simulink model "vdynblksskidpad_final"  (R2026b)
settings: Solver=ode23t  StopTime=inf  RelTol=5e-3
model workspace (MAT data in the model file):
  Eng : object (value not decoded)
  Nmtr = 11.5
  StartupTrim : object (value not decoded)
  SteerLim = 60
  TrackPoints = [-15 -12 -9 -6 -3 5.58745102111e-16 2.81978007367 5.36354042717 7.38228007367 8.67839071119 9.125 8.67839071119 ... (270 elements, 90x3)]
  Trans : object (value not decoded)
  Ts = 0.02
  VEH : object (value not decoded)
values from neighbouring files (symbols this model uses):
  n = size(e.Data,2)    [plot_skidpad_signals.m]
  z = tsMatrix(out.diagWheel.z)    [skidpad_settle_start.m]
symbols that are objects in the model workspace (value not decoded): Eng, StartupTrim, Trans, VEH
undefined symbols (not defined in the file or in its folder): BdyFrm, InertFrm, magnitude
libraries: autolibsharedcoupling x11, simulink x8, sim3dlib x7, autolibshareddiff x5, autolibutils x4, sim3dautolib x3, vehdynlibtirecommon x3, sharedtransform x3, vehdynlibdriver x2, vehdynlibsteering x2, vehdynlibeom x2, vehdynlibviscommon x2
(part 2 of 5)

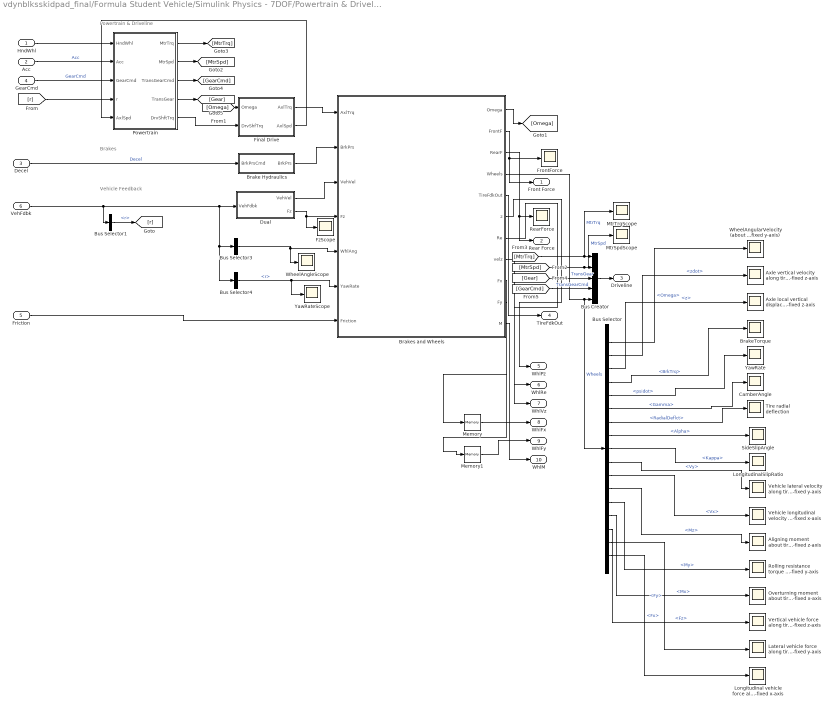
== system vdynblksskidpad_final/Formula Student Vehicle/Simulink Physics - 7DOF/Powertrain & Driveline ==
  note: Brakes
  note: Powertrain & Driveline
  note: Vehicle Feedback
  HndWhl : Inport
  Acc : Inport  Port=2
  Decel : Inport  Port=3
  GearCmd : Inport  Port=4
  Friction : Inport  Port=5
  VehFdbk : Inport  Port=6
  Aligning moment about tire-fixed z-axis : Scope
      settings: DataLoggingVariableName=ScopeData27
  "Axle local vertical displacement along tire-fixed z-axis " : Scope
      settings: DataLoggingVariableName=ScopeData18
  Axle vertical velocity along tire-fixed z-axis : Scope
      settings: DataLoggingVariableName=ScopeData17
  Brake Hydraulics : Subsystem
  BrakeTorque : Scope
      settings: DataLoggingVariableName=ScopeData19
  Brakes and Wheels : Subsystem
      mask Display: image('vdbslibwhls.png');
  Bus Creator : BusCreator  Inputs=5
  Bus Selector : BusSelector  OutputSignals=Omega,zdot,z,BrkTrq,psidot,Gamma,RadialDeflct,Alpha,Kappa,Vy,Vx,Mz,My,Mx,Fz,Fy,Fx
  Bus Selector1 : BusSelector  OutputSignals=signal1.VehFdbk.BdyFrm.Cg.AngVel.r
  Bus Selector3 : BusSelector  OutputSignals=signal2  OutputAsBus=on
  Bus Selector4 : BusSelector  OutputSignals=signal1.VehFdbk.BdyFrm.Cg.AngVel.r
  CamberAngle : Scope
      settings: DataLoggingVariableName=ScopeData21
  Dual : Subsystem  VariantControl=1
  Final Drive : Subsystem  Variant=on  VariantControlMode=label  VariantControl=Variant1  LabelModeActiveChoice=Direct
  FrontForce : Scope
      settings: ActiveDisplayYMinimum=-5430.7562675409335  ActiveDisplayYMaximum=5616.5134549978548  DataLoggingVariableName=ScopeData6
  FzScope : Scope
      settings: ActiveDisplayYMinimum=-645.63329923322237  ActiveDisplayYMaximum=1662.7938538455548  DataLoggingVariableName=ScopeData8
  Lateral vehicle force along tire-fixed y-axis : Scope
      settings: DataLoggingVariableName=ScopeData31
  Longitudinal vehicle force along tire-fixed x-axis : Scope
      settings: DataLoggingVariableName=ScopeData32
  LongitudinalSlipRatio : Scope
      settings: DataLoggingVariableName=ScopeData24
  Memory : Memory
  Memory1 : Memory
  MtrSpdScope : Scope
      settings: ActiveDisplayYMinimum=-7990.9819579860705  ActiveDisplayYMaximum=10917.06072261999  DataLoggingVariableName=ScopeData5
  MtrTrqScope : Scope
      settings: ActiveDisplayYMinimum=-20.850315998209098  ActiveDisplayYMaximum=27.207842066624828  DataLoggingVariableName=ScopeData4
  "Overturning moment about tire-fixed x-axis " : Scope
      settings: DataLoggingVariableName=ScopeData29
  Powertrain : Subsystem  Variant=on  VariantControlMode=label  VariantControl=Powertrain  LabelModeActiveChoice=EV4EM  EmptyChoice=on
  RearForce : Scope
      settings: ActiveDisplayYMinimum=-3774.7383769148314  ActiveDisplayYMaximum=3034.9269366821081  DataLoggingVariableName=ScopeData7
  Rolling resistance torque about tire-fixed y-axis : Scope
      settings: DataLoggingVariableName=ScopeData28
  SideSlipAngle : Scope
      settings: ActiveDisplayYMinimum=-0.025723950583025436  ActiveDisplayYMaximum=-0.012444025446734935  DataLoggingVariableName=ScopeData23
  Tire radial deflection : Scope
      settings: DataLoggingVariableName=ScopeData22
  Vehicle lateral velocity along tire-fixed y-axis : Scope
      settings: DataLoggingVariableName=ScopeData25
  Vehicle longitudinal velocity along tire-fixed x-axis : Scope
      settings: ActiveDisplayYMinimum=-9.3486138693816443  ActiveDisplayYMaximum=18.874913708365771  DataLoggingVariableName=ScopeData26
  Vertical vehicle force along tire-fixed z-axis : Scope
      settings: DataLoggingVariableName=ScopeData30
  WheelAngleScope : Scope
      settings: ActiveDisplayYMinimum=-1.4321699263684977  ActiveDisplayYMaximum=0.32820753202327618  DataLoggingVariableName=ScopeData10
  WheelAngularVelocity (about wheel-fixed y-axis) : Scope
      settings: ActiveDisplayYMinimum=-103.38838312860861  ActiveDisplayYMaximum=88.850056409744354  DataLoggingVariableName=ScopeData16
  YawRate : Scope
      settings: DataLoggingVariableName=ScopeData20
  YawRateScope : Scope
      settings: ActiveDisplayYMinimum=-2.8485480894872084  ActiveDisplayYMaximum=2.5377303717967763  DataLoggingVariableName=ScopeData9
  Front Force : Outport  VectorParamsAs1DForOutWhenUnconnected=off
  Rear Force : Outport  Port=2  VectorParamsAs1DForOutWhenUnconnected=off
  Driveline : Outport  Port=3  VectorParamsAs1DForOutWhenUnconnected=off
  TireFdkOut : Outport  Port=4
  WhlPz : Outport  Port=5
  WhlRe : Outport  Port=6
  WhlVz : Outport  Port=7
  WhlFx : Outport  Port=8
  WhlFy : Outport  Port=9
  WhlM : Outport  Port=10
  wires:
  [Omega] -> Final Drive/1(Omega)
  Decel/1 -> Brake Hydraulics/1(BrkPrsCmd)  "Decel"
  Friction/1 -> Brakes and Wheels/7(Friction)
  VehFdbk/1 -> Bus Selector1/1, Dual/1(VehFdbk), Bus Selector4/1, Bus Selector3/1
  Brakes and Wheels/1(Omega) -> [Omega]
  Brakes and Wheels/2(FrontF) -> Front Force/1, FrontForce/1
  Brakes and Wheels/3(RearF) -> Rear Force/1, RearForce/1
  Bus Selector3/1 -> WheelAngleScope/1, Brakes and Wheels/5(WhlAng)
  Bus Selector4/1 -> Brakes and Wheels/6(YawRate), YawRateScope/1  "<r>"
  Brake Hydraulics/1(BrkPrs) -> Brakes and Wheels/2(BrkPrs)
  Final Drive/1(AxlTrq) -> Brakes and Wheels/1(AxlTrq)
  Dual/1(VehVel) -> Brakes and Wheels/3(VehVel)
  Brakes and Wheels/4(Wheels) -> Bus Selector/1, Bus Creator/5  "Wheels"
  Bus Creator/1 -> Driveline/1
  [MtrSpd] -> MtrSpdScope/1, Bus Creator/2  "MtrSpd"
  [MtrTrq] -> MtrTrqScope/1, Bus Creator/1  "MtrTrq"
  [Gear] -> Bus Creator/3  "TransGear"
  [GearCmd] -> Bus Creator/4  "TransGearCmd"
  Dual/2(Fz) -> FzScope/1, Brakes and Wheels/4(Fz)
  Acc/1 -> Powertrain/2(Acc)  "Acc"
  GearCmd/1 -> Powertrain/3(GearCmd)  "GearCmd"
  Final Drive/2(AxlSpd) -> Powertrain/5(AxlSpd)
  Powertrain/1(MtrTrq) -> [MtrTrq]
  Powertrain/2(MtrSpd) -> [MtrSpd]
  Powertrain/3(TransGearCmd) -> [GearCmd]
  Powertrain/4(TransGear) -> [Gear]
  Powertrain/5(DrvShftTrq) -> Final Drive/2(DrvShfTrq)
  HndWhl/1 -> Powertrain/1(HndWhl)
  Bus Selector1/1 -> [r]  "<r>"
  [r] -> Powertrain/4(r)
  Brakes and Wheels/5(TireFdkOut) -> TireFdkOut/1
  Bus Selector/1 -> WheelAngularVelocity (about wheel-fixed y-axis)/1  "<Omega>"
  Bus Selector/2 -> Axle vertical velocity along tire-fixed z-axis/1  "<zdot>"
  Bus Selector/3 -> "Axle local vertical displacement along tire-fixed z-axis "/1  "<z>"
  Bus Selector/4 -> BrakeTorque/1  "<BrkTrq>"
  Bus Selector/5 -> YawRate/1  "<psidot>"
  Bus Selector/6 -> CamberAngle/1  "<Gamma>"
  Bus Selector/7 -> Tire radial deflection/1  "<RadialDeflct>"
  Bus Selector/8 -> SideSlipAngle/1  "<Alpha>"
  Bus Selector/9 -> LongitudinalSlipRatio/1  "<Kappa>"
  Bus Selector/10 -> Vehicle lateral velocity along tire-fixed y-axis/1  "<Vy>"
  Bus Selector/11 -> Vehicle longitudinal velocity along tire-fixed x-axis/1  "<Vx>"
  Bus Selector/12 -> Aligning moment about tire-fixed z-axis/1  "<Mz>"
  Bus Selector/13 -> Rolling resistance torque about tire-fixed y-axis/1  "<My>"
  Bus Selector/14 -> "Overturning moment about tire-fixed x-axis "/1  "<Mx>"
  Bus Selector/15 -> Vertical vehicle force along tire-fixed z-axis/1  "<Fz>"
  Bus Selector/16 -> Lateral vehicle force along tire-fixed y-axis/1  "<Fy>"
  Bus Selector/17 -> Longitudinal vehicle force along tire-fixed x-axis/1  "<Fx>"
  Brakes and Wheels/6(z) -> WhlPz/1
  Brakes and Wheels/7(Re) -> WhlRe/1
  Brakes and Wheels/8(velz) -> WhlVz/1
  Brakes and Wheels/9(Fx) -> Memory/1
  Brakes and Wheels/10(Fy) -> Memory1/1
  Brakes and Wheels/11(M) -> WhlM/1
  Memory/1 -> WhlFx/1
  Memory1/1 -> WhlFy/1

== system vdynblksskidpad_final/Formula Student Vehicle/Simulink Physics - 7DOF/Steering ==
  HndWhl : Inport
  TireFdkIn : Inport  Port=2
  VehSpd : Inport  Port=3
  AngLftScope : Scope
      settings: ActiveDisplayYMinimum=-1.2216121403987263  ActiveDisplayYMaximum=0.8082696461676675  DataLoggingVariableName=ScopeData2
  AngRghtScope : Scope
      settings: ActiveDisplayYMinimum=-3.9130000884146967  ActiveDisplayYMaximum=5.4341187455703839
  Constant : Constant  Commented=on  Value=[2.6, 2.6]  VectorParams1D=off
  Degrees to Radians : simulink_extras/Transformations/Degrees to Radians  Commented=on
  Kinematic Steering : vehdynlibsteering/Kinematic Steering  StrgType=Ackerman  StrgRatioType=Constant  Loc=Front  NrmlFctr=1  TrckWdth=1.2  WhlBase=1.55  Db=0  StrgRng=2*pi/3  StrgAngBpts="[-6.2832   -5.0265   -3.7699   -2.5133   -1.2566         0    1.2566    2.5133    3.7699    5.0265    6.2832]"  StrgRatioTbl=|  StrgRatio=4.67  PctAckIn=off  PctAck=92  PctAckTbl=ones(1,11)*100  StrgArmLngth=0.1  RckCsLngth=0.5  TieRodLngth=0.248128028933392  D=0.2  PnnRadius=0.0057  PnnRadiusTbl="[0.0055    0.0055    0.0056    0.0057    0.0057    0.0057    0.0057    0.0057    0.0056    0.0055    0.0055]"  RodLngth=0.1  ParaArmLngth=0.9  aMode=2
      | [13.5000   13.3750   13.2500   13.1250   13.0000   13.0000   13.0000   13.1250   13.2500   13.3750   13.5000
      | ]
  Mux : Mux  Inputs=2
  Normalized Steering : Gain  Gain=SteerLim*pi/180*10
  Reshape : Reshape  Commented=on  OutputDimensionality=Customize  OutputDimensions=[1,2]
  Steering System : vehdynlibsteering/Steering System  Commented=on  StrgType=Rack and pinion  IntmdShaftType=Double Cardan joints  PwrAst=on  AckStr=on  PwrAstOverride=off  AckStrOverride=off  KingpinOverride=off  Loc=Front  StrIn=Angle  TrckWdth=1.2  WhlBase=1.55  StrRng=1.5*pi  DbWdth=0  StrWhlInert=0.1  StrColInert=0.01  KngpnOfst=0.075  Lambda=0.2094  HbLead=4.00E-05  StcLdRadius=0.4  OvrlStrRatio=4.67  StrgAngBpts="[-6.2832   -5.0265   -3.7699   -2.5133   -1.2566         0    1.2566    2.5133    3.7699    5.0265    6.2832]"  CstrAng=0  StrgRatioType=Constant  RckGn=0.087  RckGnTbl=ones(1,11)*0.0057*2*pi  RckPnAlgm=Kinematics  RackDispBpts=[-40 -19.2 -4.53 4.53 19.2 40]  RghtWhlAngTbl=[-1.5*pi -0.72*pi -0.17*pi 0.17*pi 0.72*pi 1.5*pi]/13.5  RghtWhlStrSpdTbl=[0.008726624950158,0.008727065906090,0.008727190569212,0.008727190569212,0.008727065906090,0.008726624950158]  LftWhlAngTbl=[-1.5*pi -0.72*pi -0.17*pi 0.17*pi 0.72*pi 1.5*pi]/13.5  LftWhlStrSpdTbl=[0.008726624950158,0.008727065906090,0.008727190569212,0.008727190569212,0.008727065906090,0.008726624950158]  StrgArmLngth=0.035  RckCsLngth=0.38  TieRodLngth=0.355  Dst=0.048  Epsilon=0.9  PnInert=0.1  SptlAng=2.6178  Alpha_b=2.6178  Alpha_c=2.7051  Sigma_bc=0.2618  Gamma=0.2618  TrqBpts=[-100 0 100]  VehSpdBpts=[0 20]  TrqTbl=[0 -100;0 0;0 100]  TrqLmt=100  PwrLmt=1000  Eta=1  omega_c=200  AckParamType=Constant  PctAck=92  PctAckTbl=ones(1,11)*100  SlgStf=1.5e4  UpprFric=1  PrsFric=1e-5  MaxStf=10000  MaxUpprFric=0.2  MaxDamp=1  TorStf=30  TorDamp=1  A=0  D=0  I=0  OutSatLowLmt=-500  OutSatUpLmt=500  P=1000
  Terminator6 : Terminator
  Vector Concatenate : Concatenate  Commented=on
  Vector Concatenate1 : Concatenate  Mode=Multidimensional array  ConcatenateDimension=2
  FrntWhl : Outport  VectorParamsAs1DForOutWhenUnconnected=off
  StrngAng : Outport  Port=2
  wires:
  Kinematic Steering/1 -> Terminator6/1
  Mux/1 -> FrntWhl/1
  HndWhl/1 -> Normalized Steering/1
  Normalized Steering/1 -> Kinematic Steering/1, Steering System/5
  Constant/1 -> Degrees to Radians/1
  Vector Concatenate/1 -> Reshape/1
  Steering System/2 -> Vector Concatenate/1
  Steering System/3 -> Vector Concatenate/2
  Kinematic Steering/2 -> Vector Concatenate1/1, AngLftScope/1, Mux/1
  Kinematic Steering/3 -> Mux/2, Vector Concatenate1/2, AngRghtScope/1
  Degrees to Radians/1 -> Steering System/1
  Reshape/1 -> Steering System/2
  TireFdkIn/1 -> Steering System/3
  VehSpd/1 -> Steering System/4
  Vector Concatenate1/1 -> StrngAng/1

== system vdynblksskidpad_final/Formula Student Vehicle/Simulink Physics - 7DOF/VehP formatter ==
  In1 : Inport
  VehP in : BusSelector  OutputSignals=InertFrm.FrntAxl.Lft.Disp.X,InertFrm.FrntAxl.Lft.Disp.Y,InertFrm.FrntAxl.Lft.Disp.Z,InertFrm.FrntAxl.Rght.Disp.X,InertFrm.FrntAxl.Rght.Disp.Y,InertFrm.FrntAxl.Rght.Disp.Z,InertFrm.RearAxl.Lft.Disp.X,InertFrm.RearAxl.Lft.Disp.Y,InertFrm.RearAxl.Lft.Disp.Z,InertFrm.RearAxl.Rght.Disp.X,InertFrm.RearAxl.Rght.Disp.Y,InertFrm.RearAxl.Rght.Disp.Z
  "VehP in 3x4 " : Concatenate  NumInputs=3  Mode=Multidimensional array
  Xp in : Concatenate  NumInputs=4  Mode=Multidimensional array  ConcatenateDimension=2
  Yp in1 : Concatenate  NumInputs=4  Mode=Multidimensional array  ConcatenateDimension=2
  Zp in1 : Concatenate  NumInputs=4  Mode=Multidimensional array  ConcatenateDimension=2
  Out1 : Outport
  wires:
  In1/1 -> VehP in/1
  Xp in/1 -> "VehP in 3x4 "/1
  VehP in/7 -> Xp in/3  "<X>"
  VehP in/1 -> Xp in/1  "<X>"
  VehP in/6 -> Zp in1/2  "<Z>"
  VehP in/3 -> Zp in1/1  "<Z>"
  VehP in/2 -> Yp in1/1  "<Y>"
  VehP in/4 -> Xp in/2  "<X>"
  VehP in/12 -> Zp in1/4  "<Z>"
  VehP in/11 -> Yp in1/4  "<Y>"
  VehP in/8 -> Yp in1/3  "<Y>"
  Yp in1/1 -> "VehP in 3x4 "/2
  VehP in/10 -> Xp in/4  "<X>"
  VehP in/5 -> Yp in1/2  "<Y>"
  Zp in1/1 -> "VehP in 3x4 "/3
  "VehP in 3x4 "/1 -> Out1/1
  VehP in/9 -> Zp in1/3  "<Z>"

== system vdynblksskidpad_final/Formula Student Vehicle/Simulink Physics - 7DOF/VehV formatter ==
  In1 : Inport
  VehV in : BusSelector  OutputSignals=InertFrm.FrntAxl.Lft.Vel.Xdot,InertFrm.FrntAxl.Lft.Vel.Ydot,InertFrm.FrntAxl.Lft.Vel.Zdot,InertFrm.FrntAxl.Rght.Vel.Xdot,InertFrm.FrntAxl.Rght.Vel.Ydot,InertFrm.FrntAxl.Rght.Vel.Zdot,InertFrm.RearAxl.Lft.Vel.Xdot,InertFrm.RearAxl.Lft.Vel.Ydot,InertFrm.RearAxl.Lft.Vel.Zdot,InertFrm.RearAxl.Rght.Vel.Xdot,InertFrm.RearAxl.Rght.Vel.Ydot,InertFrm.RearAxl.Rght.Vel.Zdot
  "VehV in 3x4 " : Concatenate  NumInputs=3  Mode=Multidimensional array
  Xv in : Concatenate  NumInputs=4  Mode=Multidimensional array  ConcatenateDimension=2
  Yv in : Concatenate  NumInputs=4  Mode=Multidimensional array  ConcatenateDimension=2
  Zv in : Concatenate  NumInputs=4  Mode=Multidimensional array  ConcatenateDimension=2
  Out1 : Outport
  wires:
  VehV in/5 -> Yv in/2  "<Ydot>"
  VehV in/11 -> Yv in/4  "<Ydot>"
  VehV in/12 -> Zv in/4  "<Zdot>"
  Xv in/1 -> "VehV in 3x4 "/1
  In1/1 -> VehV in/1
  VehV in/9 -> Zv in/3  "<Zdot>"
  VehV in/7 -> Xv in/3  "<Xdot>"
  Zv in/1 -> "VehV in 3x4 "/3
  VehV in/4 -> Xv in/2  "<Xdot>"
  "VehV in 3x4 "/1 -> Out1/1
  VehV in/6 -> Zv in/2  "<Zdot>"
  VehV in/1 -> Xv in/1  "<Xdot>"
  VehV in/2 -> Yv in/1  "<Ydot>"
  Yv in/1 -> "VehV in 3x4 "/2
  VehV in/10 -> Xv in/4  "<Xdot>"
  VehV in/3 -> Zv in/1  "<Zdot>"
  VehV in/8 -> Yv in/3  "<Ydot>"

== system vdynblksskidpad_final/Formula Student Vehicle/Simulink Physics - 7DOF/Vehicle Body 3DOF Dual Track ==
  WhlAngF : Inport
  FwF : Inport  Port=2
  FwR : Inport  Port=3
  Add : Sum
  FrontAxleNormalForce : Scope
      settings: ActiveDisplayYMinimum=-1242.579827063583  ActiveDisplayYMaximum=3431.5629429130913  DataLoggingVariableName=ScopeData14
  RearAxleNormalForce : Scope
      settings: DataLoggingVariableName=ScopeData15
  Sqrt : Sqrt
  Square : Math  Operator=square
  Square1 : Math  Operator=square
  Terminator{2..4,7} (4 alike) : Terminator
  Vehicle Body 3DOF Dual Track : autolibshared/Vehicle Body 3DOF Single Track  trackMode=Dual  inputMode=External forces  frontSteerMode=on  rearSteerMode=off  extFMode=off  htchFMode=off  extMMode=off  htchMMode=off  windMode=off  extTamb=off  muMode=off  extGndPlnElev=off  extGndPlnRoll=off  extGndPlnPitch=off  extGndPlnDCM=off  extXo=off  extxdoto=off  extYo=off  extydoto=off  extpsio=off  extro=off  aMode=2  NF=2  NR=2  m=258  a=1.55*0.55  b=1.55*0.45  h=0.3/2  dh=1  hh=0.2  X_o=VEH.InitialLongPosition  xdot_o=VEH.InitialLongVel  d=0  hl=0  w=1.2*[1 1.25/1.2]  CalphaMode=Constant  sigmaMode=on  sigma_f=.1  sigma_r=.1  Cy_f=15000  Cy_r=35000  Cy_f_data=[2000, 3000, 4000, 5500, 7000, 9000, 7000, 5500, 4000, 3000, 2000]  alpha_f_brk=[-.1 .1]  Fz_f_brk="[500\t1.555555555555556e+03\t2.611111111111111e+03\t3.666666666666667e+03\t4.722222222222223e+03\t5.777777777777777e+03\t6.833333333333333e+03\t7.888888888888889e+03\t8.944444444444445e+03\t10000]"  Cy_r_data=[2000, 3000, 4000, 5500, 7000, 9000, 7000, 5500, 4000, 3000, 2000]  alpha_r_brk=[-.1 .1]  Fz_r_brk="[500\t1.555555555555556e+03\t2.611111111111111e+03\t3.666666666666667e+03\t4.722222222222223e+03\t5.777777777777777e+03\t6.833333333333333e+03\t7.888888888888889e+03\t8.944444444444445e+03\t10000]"  Fznom=3800  Y_o=VEH.InitialLatPosition  ydot_o=VEH.InitialLatVel  Izz=VEH.YawMomentInertia  psi_o=VEH.InitialYawAngle  r_o=VEH.InitialYawRate  Af=1  Cd=1.8  Cl=4.8  Cpm=.1  beta_w=[0 0.01:0.01:0.3]  Cs=[0 0.01:0.01:0.3]  Cym=[0 1e-6:0.01:0.3]  Pabs=101325  Tair=273  g=9.81  mu=1  GndPlnRoll=0  GndPlnPitch=0  GndPlnElev=0  xdot_tol=.01  Fxtire_sat=7e3*1e3  Fytire_sat=2e3*1e3  longOff=0  latOff=0  vertOff=.0112  wrapAng=off
  Vehicle Body 6DOF : vehdynlibeom/Vehicle Body 6DOF  extPos=on  extVel=on  extEuler=on  extRotRate=on  htchFMode=off  htchMMode=off  m=2000  a=1.4  b=1.6  d=0  h=0.35  dh=1  hl=0  hh=0.1  Xe_o=[0,0,0]  xbdot_o=[0,0,0]  eul_o=[0,0,0]  p_o=[0,0,0]  Iveh=[430 0 0; 0 1900 0; 0 0 2100]  w=[1.9,1.9]  z1m=0  z1R=[.25,.125,-0.15]  z1I=[1.4,-.2,.1;-.2,1.4,.1;.1,.1,2.25].*0  z2m=0  z2R=[-1.4,0,-0.8]  z2I=[1.4,-.2,.1;-.2,1.4,.1;.1,.1,2.25].*0  z3m=0  z3R=[-.75,-0.5,-0.4]  z3I=[5,-.1,-2;-2,9,.1;-.1,.1,6].*0  z4m=0  z4R=[-.75,.5,-0.4]  z4I=[5,-.1,-2;-2,9,.1;-.1,.1,6].*0  z5m=0  z5R=[-1.25,-.5,-0.4]  z5I=[5,-.1,-2;-2,9,.1;-.1,.1,6].*0  z6m=0  z6R=[-1.25,0.5,-0.4]  z6I=[5,-.1,-2;-2,9,.1;-.1,.1,6].*0  z7m=0  z7R=[-2,0,-0.25]  z7I=[1.4,-.2,.1;-.2,1.4,.1;.1,.1,2.25].*0  Af=2  Cd=.3  Cl=.1  Cpm=.1  beta_w=[0:0.001:0.01]  Cs=[0:0.01:0.1]  Cym=[0:0.001:0.01]  Pabs=101325  extTamb=off  Tair=273  g=9.81  xdot_tol=.1  longOff=0  latOff=0  vertOff=0.35  wrapAng=on  aMode=2
  VehicleSpeedScope : Scope
      settings: DataLoggingVariableName=ScopeData11
  YawRateScope : Scope
      settings: DataLoggingVariableName=ScopeData13
  YawScope : Scope
      settings: DataLoggingVariableName=ScopeData12
  VehFdbk : Outport
  VehVel : Outport  Port=2
  wires:
  Vehicle Body 3DOF Dual Track/6 -> FrontAxleNormalForce/1, Terminator3/1
  Vehicle Body 3DOF Dual Track/2 -> Square/1
  Vehicle Body 3DOF Dual Track/3 -> Square1/1
  Vehicle Body 3DOF Dual Track/4 -> YawScope/1, Terminator2/1
  Vehicle Body 3DOF Dual Track/7 -> RearAxleNormalForce/1, Terminator4/1
  Vehicle Body 3DOF Dual Track/1 -> VehFdbk/1  "VehFdbk"
  Vehicle Body 3DOF Dual Track/5 -> YawRateScope/1, Terminator7/1
  FwF/1 -> Vehicle Body 3DOF Dual Track/2
  WhlAngF/1 -> Vehicle Body 3DOF Dual Track/1
  FwR/1 -> Vehicle Body 3DOF Dual Track/3
  Square/1 -> Add/1
  Square1/1 -> Add/2
  Add/1 -> Sqrt/1
  Sqrt/1 -> VehicleSpeedScope/1, VehVel/1

== system vdynblksskidpad_final/Formula Student Vehicle/Simulink Physics - 7DOF/Velocity to Speed ==
  In1 : Inport
  Bus Selector3 : BusSelector  OutputSignals=InertFrm.Cg.Vel.Xdot,InertFrm.Cg.Vel.Ydot,InertFrm.Cg.Vel.Zdot
  Magnitude Squared : Math  Operator=magnitude^2
  Magnitude Squared1 : Math  Operator=magnitude^2
  Magnitude Squared2 : Math  Operator=magnitude^2
  Sum : Sum  Inputs=|+++
  Out1 : Outport
  wires:
  In1/1 -> Bus Selector3/1
  Bus Selector3/1 -> Magnitude Squared/1  "<Xdot>"
  Magnitude Squared/1 -> Sum/1
  Sum/1 -> Out1/1
  Bus Selector3/2 -> Magnitude Squared1/1  "<Ydot>"
  Magnitude Squared1/1 -> Sum/2
  Magnitude Squared2/1 -> Sum/3
  Bus Selector3/3 -> Magnitude Squared2/1  "<Zdot>"

== system vdynblksskidpad_final/Visualization/3D Visualization/Disabled ==

== system vdynblksskidpad_final/Visualization/3D Visualization/Enabled ==
  VehFdbk : Inport
  3D Visualization : Subsystem  Variant=on  VariantControl=Choice
  Cones : Subsystem  Variant=on  VariantControl=Choice
  wires:
  VehFdbk/1 -> 3D Visualization/1(VehFdbk)

== system vdynblksskidpad_final/Formula Student Vehicle/Simulink Physics - 7DOF/Environment/Ground Feedback ==
  note: 1) Add Subsystem or Model blocks as valid variant choices.
      | 2) You cannot connect blocks at this level. At simulation, connectivity is automatically
      | determined, based on the active variant and port name matching.
  Friction : Inport
  Constant : Subsystem  VariantControl=0
  Ground : Outport  VectorParamsAs1DForOutWhenUnconnected=off

== system vdynblksskidpad_final/Formula Student Vehicle/Simulink Physics - 7DOF/Powertrain & Driveline/Brake Hydraulics ==
  BrkPrsCmd : Inport
  Dead Zone : DeadZone  LowerValue=-inf  UpperValue=1e-3  ZeroCross=off
  Front Bias : Constant
  Gain4 : Gain  Gain=1e6
  Mux : Mux
  Product : Product
  Rear Bias : Constant  Value=.6
  Selector : Selector  InputPortWidth=1  IndexOptions=Index vector (dialog)  Indices=[1 1 1 1]  OutputSizes=1  RuntimeRangeChecks=off
  Valve : autolibutils/Cont LPF  wc=40*pi  AbsoluteTolerance=auto  aMode=2
  BrkPrs : Outport  VectorParamsAs1DForOutWhenUnconnected=off
  wires:
  BrkPrsCmd/1 -> Valve/1
  Valve/1 -> Dead Zone/1  "Flow"
  Gain4/1 -> BrkPrs/1
  Front Bias/1 -> Mux/2, Mux/1
  Rear Bias/1 -> Mux/3, Mux/4
  Product/1 -> Gain4/1
  Mux/1 -> Product/1
  Selector/1 -> Product/2
  Dead Zone/1 -> Selector/1

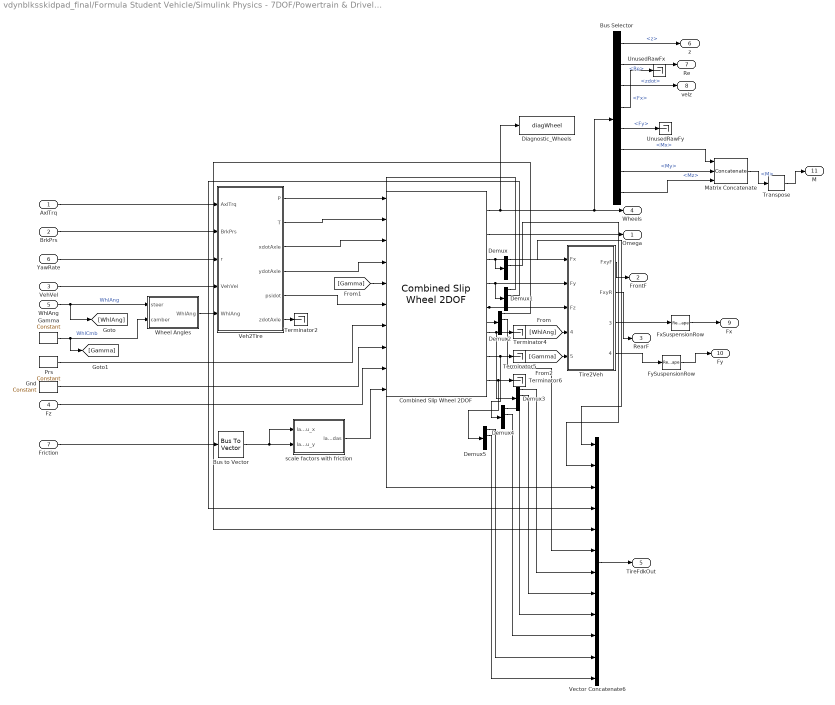
== system vdynblksskidpad_final/Formula Student Vehicle/Simulink Physics - 7DOF/Powertrain & Driveline/Brakes and Wheels ==
  AxlTrq : Inport
  BrkPrs : Inport  Port=2
  VehVel : Inport  Port=3
  Fz : Inport  Port=4  PortDimensions=4
  WhlAng : Inport  Port=5
  YawRate : Inport  Port=6
  Friction : Inport  Port=7
  Bus Selector : BusSelector  OutputSignals=z,Re,zdot,Fx,Fy,Mx,My,Mz
  Bus to Vector : BusToVector
  Combined Slip Wheel 2DOF : vehdynlibtire/Combined Slip Wheel 2DOF  tireType=External file  tireParamSet=/Users/aaditya/Desktop/VD_Racing_Team/FSAE_16_inch_new_converted_to_MF62.tir  scaleFactorInput=on  vertType=Magic Formula  plySteer=off  turnslip=on  BrakeType=Disc  mu_static=.3  mu_kinetic=.2  drum_abore=0.0508  drum_a=0.123  drum_c=0.212  drum_r=0.15  drum_theta1=0  drum_theta2=126  disk_abore=.05  Rm=.177  num_pads=2  brake_p_bpt=[1 11.4736842105263 21.9473684210526 32.4210526315789 42.8947368421053 53.3684210526316 63.8421052631579 74.3157894736842 84.7894736842105 95.2631578947368 105.736842105263 116.210526315789 126.684210526316 137.157894736842 147.631578947368 158.105263157895 168.578947368421 179.052631578947 189.526315789474 200]  brake_n_bpt=[0 52.6315789473684 105.263157894737 157.894736842105 210.526315789474 263.157894736842 315.789473684211 368.421052631579 421.052631578947 473.684210526316 526.315789473684 578.947368421053 631.578947368421 684.210526315789 736.842105263158 789.473684210526 842.105263157895 894.736842105263 947.368421052632 1000]  f_brake_t=[43.4900602404453 42.5056030554862 41.5350898940194 40.5780454442085 39.6340111501808 38.7025443887544 37.7832176914519 36.8756180088306 35.9793460143796 35.0940154454303 34.2192524787115 33.3546951383474 32.4999927342521 31.6548053290159 30.8188032315107 29.991666515561 29.1730845621415 28.362755623661 27.5603864089927 26.765691687993;498.991217495636 487.695866636631 476.560505099801 465.579679307235 454.748127933653 444.060772460445 433.51270824929 423.099196101319 412.81565427025 402.657650900201 392.620896861006 382.701238955775 372.894653477208 363.197240090814 353.605216024701 344.114910546964 334.722759712992 325.425301366216 316.219170376863 307.10109410434;954.492374750826 932.886130217776 911.585920305583 890.581313170261 869.862244717126 849.419000532136 829.242198807128 809.322774193808 789.651962526121 770.221286354971 751.0225412433 732.047782773203 713.289314220164 694.739674852612 676.391628817892 658.238154578366 640.272434863842 622.48784710877 604.877954344734 587.436496520688;1409.99353200602 1378.07639379892 1346.61133551136 1315.58294703329 1284.9763615006 1254.77722860383 1224.97168936497 1195.5463522863 1166.48827078199 1137.78492180974 1109.42418562559 1081.39432659063 1053.68397496312 1026.28210961441 999.178041611083 972.361398609768 945.822110014692 919.550392851325 893.536738312604 867.771898937035;1865.49468926121 1823.26665738007 1781.63675071715 1740.58458089631 1700.09047828407 1660.13545667552 1620.7011799228 1581.76993037878 1543.32457903786 1505.34855726451 1467.82583000789 1430.74087040806 1394.07863570608 1357.82454437621 1321.96445440427 1286.48464264117 1251.37178516554 1216.61293859388 1182.19552228048 1148.10730135338;2320.9958465164 2268.45692096121 2216.66216592293 2165.58621475934 2115.20459506754 2065.49368474721 2016.43067048064 1967.99350847127 1920.16088729373 1872.91219271928 1826.22747439018 1780.08741422549 1734.47329644903 1689.36697913801 1644.75086719747 1600.60788667257 1556.92146031639 1513.67548433643 1470.85430624835 1428.44270376973;2776.49700377159 2713.64718454235 2651.68758112871 2590.58784862237 2530.31871185102 2470.8519128189 2412.16016103848 2354.21708656376 2296.9971955496 2240.47582817405 2184.62911877248 2129.43395804292 2074.86795719199 2020.9094138998 1967.53727999066 1914.73113070398 1862.47113546724 1810.73803007899 1759.51309021622 1708.77810618608;3231.99816102678 3158.8374481235 3086.71299633449 3015.58948248539 2945.43282863449 2876.21014089059 2807.88965159632 2740.44066465625 2673.83350380547 2608.03946362882 2543.03076315477 2478.78050186034 2415.26261793494 2352.4518486616 2290.32369278385 2228.85437473538 2168.02081061809 2107.80057582154 2048.17187418409 1989.11350860242;3687.49931828197 3604.02771170464 3521.73841154027 3440.59111634842 3360.54694541796 3281.56836896228 3203.61914215416 3126.66424274874 3050.66981206134 2975.60309908359 2901.43240753707 2828.12704567777 2755.6572786779 2683.9942834234 2613.11010557704 2542.97761876678 2473.57048576894 2404.8631215641 2336.83065815196 2269.44891101877;4143.00047553716 4049.21797528579 3956.76382674606 3865.59275021144 3775.66106220143 3686.92659703397 3599.34863271199 3512.88782084123 3427.50612031721 3343.16673453836 3259.83405191936 3177.4735894952 3096.05193942085 3015.5367181852 2935.89651837023 2857.10086279818 2779.12016091979 2701.92566730665 2625.48944211983 2549.78431343512;4598.50163279235 4494.40823886693 4391.78924195184 4290.59438407447 4190.77517898491 4092.28482510566 3995.07812326983 3899.11139893372 3804.34242857308 3710.73036999313 3618.23569630166 3526.82013331263 3436.44660016381 3347.079152947 3258.68293116342 3171.22410682959 3084.66983607064 2998.98821304921 2914.1482260877 2830.11971585147;5054.00279004754 4939.59850244808 4826.81465715762 4715.59601793749 4605.88929576838 4497.64305317735 4390.80761382767 4285.3349770262 4181.17873682896 4078.2940054479 3976.63734068395 3876.16667713006 3776.84126090677 3678.62158770879 3581.46934395661 3485.34735086099 ...(+2764 chars)]  NOMPRES=70000  PRESMAX=100000  PRESMIN=45000  FNOMIN=1080  FZMAX=3000  FZMIN=200  VXLOW=1  KPUMAX=1.5  KPUMIN=-1.5  ALPMAX=0.7854  ALPMIN=-0.7854  CAMMAX=0.17453  CAMMIN=-0.17453  LONGVL=16.6  FxRelFreqLwrLim=200*pi  FyRelFreqLwrLim=200*pi  MyRelFreqLwrLim=100*pi  omegao=0  UNLOADED_RADIUS=0.2032  WIDTH=0.205  RIM_RADIUS=0.1270  ASPECT_RATIO=0.45  MASS=9.3  IYY=0.736  br=1e-3  GRAVITY=-9.81  LFZO=1  LMUX=1  LMUY=1  LMUV=0  LKX=1  LKY=1  LCX=1  LCY=1  LEX=1  LEY=1  LHX=1  LHY=1  LVX=1  LVY=1  LKYC=1  LKZC=1  LTR=1  LRES=1  LXAL=1  LYKA=1  LVYKA=1  LS=1  LCZ=1  LMX=1  LVMX=1  LMY=1  LMP=1  zo=StartupTrim.TireCompression  zdoto=0  BREFF=8.81771  DREFF=0.22874  FREFF=0.01002  Q_RE0=0.9974  Q_V1=0.00077  Q_V2=0  Q_FZ1=0  Q_FZ2=0.0476  Q_FZ3=0  Q_FCX=0  Q_FCY=0  Q_FCY2=0  PFZ1=0  VERTICAL_STIFFNESS=90000  VERTICAL_DAMPING=50  BOTTOM_OFFST=0.01  BOTTOM_STIFF=2000000  Q_CAM1=0  Q_CAM2=0  Q_CAM3=0  Q_FYS1=0  Q_FYS2=0  Q_FYS3=0  LONGITUDINAL_STIFFNESS=358066  LATERAL_STIFFNESS=174776.2  PCFX1=0.0293  PCFX2=-0.05805  PCFX3=0  PCFY1=-0.43226  PCFY2=0.06248  PCFY3=0  Q_RA1=0.671  Q_RA2=0.733  Q_RB1=1.059  Q_RB2=-1.1878  PCX1=1.4012  PDX1=2.27405  PDX2=-0.48493  PDX3=-1e-05  PEX1=-13.791  PEX2=38.727  PEX3=-17.875  PEX4=-0.5  PKX1=39.094  PKX2=-8.14679  PKX3=-0.13706  PHX1=0.0486  PHX2=0.03522  PVX1=-0.33695  PVX2=0.06631  PPX1=0  PPX2=0  PPX3=0  PPX4=0  RBX1=12.013  RBX2=10.743  RBX3=0.0132  RCX1=1.06849  REX1=-0.14817  REX2=-0.09091  RHX1=0.00636  QSX1=0  QSX2=0.00017  QSX3=0  QSX4=4.41904  QSX5=1.06344  QSX6=1.81561  QSX7=1e-05  QSX8=0  QSX9=0.55149  QSX10=0.00011  QSX11=10.687  QSX12=0  QSX13=0  QSX14=0  PPMX1=0  PCY1=1.46639  PDY1=2.29899  PDY2=-0.47709  PDY3=5.88962  PEY1=-0.21631  PEY2=-0.90056  PEY3=-0.0083  PEY4=-10  PEY5=-10  PKY1=-39.721  PKY2=0.75016  PKY3=0.88623  PKY4=2.01237  PKY5=5.4919  PKY6=-1.47864  PKY7=1.14808  PHY1=-0.00089  PHY2=-0.00055  PVY1=-0.06473  PVY2=-0.01237  PVY3=-0.54751  PVY4=0.96253  PPY1=0  PPY2=0  PPY3=0  PPY4=0  PPY5=0  RBY1=6.41916  RBY2=4.20694  RBY3=-0.01486  RBY4=0.72172  RCY1=1.08039  REY1=-0.01515  REY2=0.00061  RHY1=0.00892  RHY2=0.05304  RVY1=-0.01071  RVY2=0.01496  RVY3=-0.09226  RVY4=6.23883  RVY5=1.89521  RVY6=11.003  QSY1=0.00309  QSY2=0  QSY3=0.00346  QSY4=0.00346  QSY5=1e-05  QSY6=0  QSY7=1.00002  QSY8=0  QBZ1=7.95849  QBZ2=-0.22849  QBZ3=0.5  QBZ4=-0.00852  QBZ5=0.17782  QBZ6=0  QBZ9=20.506  QBZ10=-0.49999  QCZ1=1.17649  QDZ1=0.21562  QDZ2=-0.0227  QDZ3=0.0252  QDZ4=10.681  QDZ6=0.06217  QDZ7=-0.01673  QDZ8=0.60946  QDZ9=-0.16846  QDZ10=-1.12149  QDZ11=-0.00135  QEZ1=-3.12049  QEZ2=2.78396  QEZ3=-0.5  QEZ4=0.01889  QEZ5=-0.62135  QHZ1=0.00469  QHZ2=-0.00186  QHZ3=0.07795  QHZ4=0.0224  PPZ1=0  PPZ2=0  SSZ1=0.04348  SSZ2=-0.00446  SSZ3=0.77667  SSZ4=-0.26408  PDXP1=0  PDXP2=0  PDXP3=0  PKYP1=0  PDYP1=0  PDYP2=0  PDYP3=0  PDYP4=0  PHYP1=1  PHYP2=1  PHYP3=0  PHYP4=0  PECP1=0  PECP2=0  QDTP1=0  QCRP1=0  QCRP2=0  QBRP1=0  QDRP1=1  QDRP2=0  aMode=2
  Demux{,1..5} (6 alike) : Demux
  Diagnostic_Wheels : ToWorkspace  VariableName=diagWheel  SaveFormat=Timeseries  SampleTime=0.01
  FxSuspensionRow : Reshape  OutputDimensionality=Row vector (2-D)
  FySuspensionRow : Reshape  OutputDimensionality=Row vector (2-D)
  Gamma : vehdynlibtirecommon/Constant  const=0  numWheels=4
  Gnd : vehdynlibtirecommon/Constant  const=0  numWheels=4
  Matrix Concatenate : Concatenate  NumInputs=3  Mode=Multidimensional array  ConcatenateDimension=2
  Prs : vehdynlibtirecommon/Constant  const=2.4e5*1.1  numWheels=4
  Terminator{2,4..6} (4 alike) : Terminator
  Tire2Veh : Subsystem
  Transpose : matrix_library/Transpose
  UnusedRawFx : Terminator
  UnusedRawFy : Terminator
  Vector Concatenate6 : Concatenate  NumInputs=12
  Veh2Tire : Subsystem
  Wheel Angles : Subsystem
  scale factors with friction : Subsystem  mask{numWheels=4}
      mask prompts: numWheels "Number of wheels"
  Omega : Outport
  FrontF : Outport  Port=2
  RearF : Outport  Port=3
  Wheels : Outport  Port=4
  TireFdkOut : Outport  Port=5
  z : Outport  Port=6
  Re : Outport  Port=7
  velz : Outport  Port=8
  Fx : Outport  Port=9
  Fy : Outport  Port=10
  M : Outport  Port=11
  wires:
  Gnd/1 -> Combined Slip Wheel 2DOF/8
  Combined Slip Wheel 2DOF/2 -> Omega/1
  Combined Slip Wheel 2DOF/7 -> Demux4/1, Terminator5/1
  Combined Slip Wheel 2DOF/6 -> Demux3/1, Terminator4/1
  Fz/1 -> Combined Slip Wheel 2DOF/9
  Veh2Tire/3(xdotAxle) -> Combined Slip Wheel 2DOF/3
  Combined Slip Wheel 2DOF/8 -> Demux5/1, Terminator6/1
  Prs/1 -> Combined Slip Wheel 2DOF/7
  Veh2Tire/5(psidot) -> Combined Slip Wheel 2DOF/6
  Combined Slip Wheel 2DOF/3 -> Demux/1, Tire2Veh/1(Fx)
  Combined Slip Wheel 2DOF/4 -> Demux1/1, Tire2Veh/2(Fy)
  Combined Slip Wheel 2DOF/5 -> Tire2Veh/3(Fz), Demux2/1
  WhlAng/1 -> [WhlAng], Wheel Angles/1(steer)  "WhlAng"
  Gamma/1 -> [Gamma], Wheel Angles/2(camber)  "WhlCmb"
  Tire2Veh/1(FxyF) -> FrontF/1
  Tire2Veh/2(FxyR) -> RearF/1
  Veh2Tire/2(T) -> Combined Slip Wheel 2DOF/2
  BrkPrs/1 -> Veh2Tire/2(BrkPrs)
  AxlTrq/1 -> Veh2Tire/1(AxlTrq)
  Wheel Angles/1(WhlAng) -> Veh2Tire/5(WhlAng)
  VehVel/1 -> Veh2Tire/4(VehVel)
  Veh2Tire/6(zdotAxle) -> Terminator2/1
  Veh2Tire/1(P) -> Combined Slip Wheel 2DOF/1
  Veh2Tire/4(ydotAxle) -> Combined Slip Wheel 2DOF/4
  YawRate/1 -> Veh2Tire/3(r)
  [WhlAng] -> Tire2Veh/4(WhlAng)
  [Gamma] -> Combined Slip Wheel 2DOF/5
  [Gamma] -> Tire2Veh/5(WhlCmb)
  Friction/1 -> Bus to Vector/1
  scale factors with friction/1(lambdas) -> Combined Slip Wheel 2DOF/10
  Bus to Vector/1 -> scale factors with friction/1(lamda_mu_x), scale factors with friction/2(lamda_mu_y)
  Demux/1 -> Vector Concatenate6/1
  Demux/2 -> Vector Concatenate6/2
  Demux1/1 -> Vector Concatenate6/3
  Demux1/2 -> Vector Concatenate6/4
  Demux2/1 -> Vector Concatenate6/5
  Demux2/2 -> Vector Concatenate6/6
  Demux3/1 -> Vector Concatenate6/7
  Demux3/2 -> Vector Concatenate6/8
  Demux4/1 -> Vector Concatenate6/9
  Demux4/2 -> Vector Concatenate6/10
  Demux5/1 -> Vector Concatenate6/11
  Demux5/2 -> Vector Concatenate6/12
  Vector Concatenate6/1 -> TireFdkOut/1
  Bus Selector/1 -> z/1  "<z>"
  Bus Selector/2 -> Re/1  "<Re>"
  Bus Selector/3 -> velz/1  "<zdot>"
  Bus Selector/6 -> Matrix Concatenate/1  "<Mx>"
  Bus Selector/7 -> Matrix Concatenate/2  "<My>"
  Bus Selector/8 -> Matrix Concatenate/3  "<Mz>"
  Matrix Concatenate/1 -> Transpose/1  "<M>"
  Transpose/1 -> M/1
  Combined Slip Wheel 2DOF/1 -> Bus Selector/1, Wheels/1, Diagnostic_Wheels/1
  FySuspensionRow/1 -> Fy/1
  FxSuspensionRow/1 -> Fx/1
  Tire2Veh/3(FxVehicleAll) -> FxSuspensionRow/1
  Tire2Veh/4(FyVehicleAll) -> FySuspensionRow/1
  Bus Selector/5 -> UnusedRawFy/1  "<Fy>"
  Bus Selector/4 -> UnusedRawFx/1  "<Fx>"

== system vdynblksskidpad_final/Formula Student Vehicle/Simulink Physics - 7DOF/Powertrain & Driveline/Dual ==
  VehFdbk : Inport
  Dual Fz : Subsystem
  Dual V : Subsystem
  VehVel : Outport  VectorParamsAs1DForOutWhenUnconnected=off
  Fz : Outport  Port=2  VectorParamsAs1DForOutWhenUnconnected=off
  wires:
  Dual V/1(Out1) -> VehVel/1
  VehFdbk/1 -> Dual Fz/1(In1), Dual V/1(In1)
  Dual Fz/1(Out1) -> Fz/1

== system vdynblksskidpad_final/Formula Student Vehicle/Simulink Physics - 7DOF/Powertrain & Driveline/Final Drive ==
  Omega : Inport
  DrvShfTrq : Inport  Port=2
  All Wheel Drive : Subsystem  VariantControl=AWD
  Direct : Subsystem  VariantControl=Direct
  Front Wheel Drive : Subsystem  VariantControl=FWD
  Rear Wheel Drive : Subsystem  VariantControl=RWD
  AxlTrq : Outport  VectorParamsAs1DForOutWhenUnconnected=off
  AxlSpd : Outport  Port=2  VectorParamsAs1DForOutWhenUnconnected=off

== system vdynblksskidpad_final/Formula Student Vehicle/Simulink Physics - 7DOF/Powertrain & Driveline/Powertrain ==
  HndWhl : Inport
  Acc : Inport  Port=2
  GearCmd : Inport  Port=3
  r : Inport  Port=4
  AxlSpd : Inport  Port=5
  4EM Powertrain : Subsystem  VariantControl=EV4EM
  ICE Powertrain : Subsystem  VariantControl=ICE
  MtrTrq : Outport
  MtrSpd : Outport  Port=2
  TransGearCmd : Outport  Port=3
  TransGear : Outport  Port=4
  DrvShftTrq : Outport  Port=5

== system vdynblksskidpad_final/Visualization/3D Visualization/Enabled/3D Visualization ==
  VehFdbk : Inport
  Disabled : Subsystem  VariantControl=engine3D==1
  Ground Following : Subsystem  VariantControl=engine3D==4
  Physical Vehicle : Subsystem  VariantControl=engine3D==3
  Simulation 3D Vehicle : Subsystem  VariantControl=engine3D==2

== system vdynblksskidpad_final/Visualization/3D Visualization/Enabled/Cones ==
  Disabled : Subsystem  VariantControl=conesOn==0
  Enabled : Subsystem  VariantControl=conesOn==1

== system vdynblksskidpad_final/Formula Student Vehicle/Simulink Physics - 7DOF/Environment/Ground Feedback/Constant ==
  Friction : Inport
  Bus Creator : BusCreator  Inputs=4
  Bus Creator2 : BusCreator  Inputs=4
  Bus Creator3 : BusCreator  Inputs=2
  Constant1 : Constant  Value=zeros(4,1)
  Demux : Demux
  Demux1 : Demux
  Signal Specification : SignalSpecification  Unit=m
  Signal Specification1 : SignalSpecification  Unit=1
  Ground : Outport  VectorParamsAs1DForOutWhenUnconnected=off
  wires:
  Bus Creator3/1 -> Ground/1
  Signal Specification1/1 -> Demux1/1
  Friction/1 -> Signal Specification1/1
  Bus Creator2/1 -> Bus Creator3/2  "mu"
  Demux1/2 -> Bus Creator2/2  "mu_FR"
  Demux1/1 -> Bus Creator2/1  "mu_FL"
  Demux1/4 -> Bus Creator2/4  "mu_RR"
  Demux1/3 -> Bus Creator2/3  "mu_RL"
  Bus Creator/1 -> Bus Creator3/1  "z"
  Demux/2 -> Bus Creator/2  "G_FR_z"
  Demux/3 -> Bus Creator/3  "G_RL_z"
  Demux/1 -> Bus Creator/1  "G_FL_z"
  Demux/4 -> Bus Creator/4  "G_RR_z"
  Signal Specification/1 -> Demux/1
  Constant1/1 -> Signal Specification/1

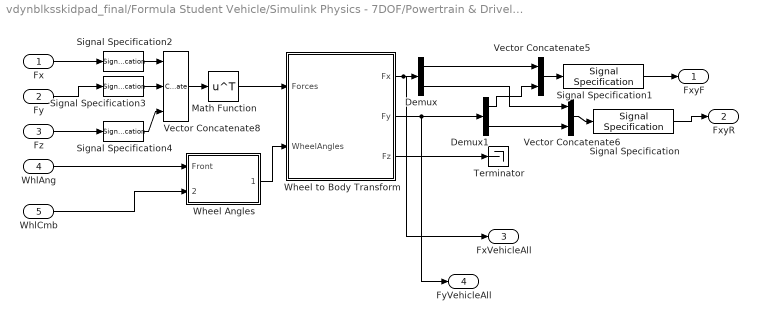
== system vdynblksskidpad_final/Formula Student Vehicle/Simulink Physics - 7DOF/Powertrain & Driveline/Brakes and Wheels/Tire2Veh ==
  Fx : Inport
  Fy : Inport  Port=2
  Fz : Inport  Port=3
  WhlAng : Inport  Port=4
  WhlCmb : Inport  Port=5
  Demux : Demux  Outputs=[2,2]
  Demux1 : Demux  Outputs=[2,2]
  Math Function : Math  Operator=transpose  SignedPower=on
  Signal Specification : SignalSpecification  Unit=N
  Signal Specification1 : SignalSpecification  Unit=N
  Signal Specification2 : SignalSpecification  Dimensions=4
  Signal Specification3 : SignalSpecification  Dimensions=4
  Signal Specification4 : SignalSpecification  Dimensions=4
  Terminator : Terminator
  Vector Concatenate5 : Concatenate  Mode=Multidimensional array  ConcatenateDimension=2
  Vector Concatenate6 : Concatenate  Mode=Multidimensional array  ConcatenateDimension=2
  Vector Concatenate8 : Concatenate  NumInputs=3  Mode=Multidimensional array  ConcatenateDimension=2
  Wheel Angles : Subsystem
  Wheel to Body Transform : Subsystem
  FxyF : Outport
  FxyR : Outport  Port=2
  FxVehicleAll : Outport  Port=3
  FyVehicleAll : Outport  Port=4
  wires:
  Vector Concatenate5/1 -> Signal Specification1/1
  Signal Specification1/1 -> FxyF/1
  Demux1/1 -> Vector Concatenate5/2
  WhlCmb/1 -> Wheel Angles/2(Camber)
  Signal Specification/1 -> FxyR/1
  Fz/1 -> Signal Specification4/1
  Fx/1 -> Signal Specification2/1
  WhlAng/1 -> Wheel Angles/1(Front)
  Signal Specification2/1 -> Vector Concatenate8/1
  Signal Specification3/1 -> Vector Concatenate8/2
  Demux/2 -> Vector Concatenate6/1
  Wheel to Body Transform/3(Fz) -> Terminator/1
  Math Function/1 -> Wheel to Body Transform/1(Forces)
  Fy/1 -> Signal Specification3/1
  Wheel to Body Transform/2(Fy) -> FyVehicleAll/1, Demux1/1
  Demux1/2 -> Vector Concatenate6/2
  Signal Specification4/1 -> Vector Concatenate8/3
  Vector Concatenate6/1 -> Signal Specification/1
  Wheel to Body Transform/1(Fx) -> FxVehicleAll/1, Demux/1
  Vector Concatenate8/1 -> Math Function/1
  Demux/1 -> Vector Concatenate5/1
  Wheel Angles/1(Vehicle) -> Wheel to Body Transform/2(WheelAngles)

== system vdynblksskidpad_final/Formula Student Vehicle/Simulink Physics - 7DOF/Powertrain & Driveline/Brakes and Wheels/Veh2Tire ==
  AxlTrq : Inport
  BrkPrs : Inport  Port=2
  r : Inport  Port=3
  VehVel : Inport  Port=4
  WhlAng : Inport  Port=5
  Reshape3 : Reshape
  Reshape4 : Reshape
  Selector : Selector  InputPortWidth=1  IndexOptions=Index vector (dialog)  Indices=[1 1 1 1]  OutputSizes=1  RuntimeRangeChecks=off
  Unary Minus : UnaryMinus
  Wheel to Body Transform : Subsystem
  P : Outport  PortDimensions=4  VectorParamsAs1DForOutWhenUnconnected=off
  T : Outport  Port=2  VectorParamsAs1DForOutWhenUnconnected=off
  xdotAxle : Outport  Port=3  PortDimensions=4  VectorParamsAs1DForOutWhenUnconnected=off
  ydotAxle : Outport  Port=4  PortDimensions=4  VectorParamsAs1DForOutWhenUnconnected=off
  psidot : Outport  Port=5  PortDimensions=4  VectorParamsAs1DForOutWhenUnconnected=off
  zdotAxle : Outport  Port=6  VectorParamsAs1DForOutWhenUnconnected=off
  wires:
  BrkPrs/1 -> Reshape3/1
  AxlTrq/1 -> Reshape4/1
  Wheel to Body Transform/1(xdotWheel) -> xdotAxle/1  "Vx"
  Wheel to Body Transform/2(ydotWheel) -> ydotAxle/1  "Vy"
  r/1 -> Unary Minus/1
  Reshape4/1 -> T/1
  VehVel/1 -> Wheel to Body Transform/1(VelVeh)
  Wheel to Body Transform/3(zdotWheel) -> zdotAxle/1  "Vz"
  Unary Minus/1 -> Selector/1
  Reshape3/1 -> P/1
  WhlAng/1 -> Wheel to Body Transform/2(WhlAng)
  Selector/1 -> psidot/1

== system vdynblksskidpad_final/Formula Student Vehicle/Simulink Physics - 7DOF/Powertrain & Driveline/Brakes and Wheels/Wheel Angles ==
  steer : Inport
  camber : Inport  Port=2
  Add1 : Sum
  Add2 : Sum
  Constant1 : Constant  Value=pi
  Constant2 : Constant  Value=[pi;0;pi;0].*0+[0;pi;0;pi].*0
  Constant3 : Constant  Value=ones(1,4).*0
  MATLAB Function : Gain  Gain=[0 0 1]  Multiplication=Matrix(K*u)
  Reshape : Reshape  OutputDimensionality=Row vector (2-D)
  Reshape1 : Reshape  OutputDimensionality=Row vector (2-D)
  Reshape2 : Reshape  OutputDimensionality=Row vector (2-D)
  Vector Concatenate3 : Concatenate  NumInputs=3  Mode=Multidimensional array
  WhlAng : Outport  VectorParamsAs1DForOutWhenUnconnected=off
  wires:
  Constant1/1 -> Add2/2
  Add2/1 -> Reshape1/1
  Add1/1 -> Reshape/1
  Reshape2/1 -> Vector Concatenate3/2
  Reshape1/1 -> Vector Concatenate3/1
  Constant3/1 -> Reshape2/1
  camber/1 -> Add2/1
  Reshape/1 -> Vector Concatenate3/3
  Vector Concatenate3/1 -> WhlAng/1
  Constant2/1 -> Add1/2
  steer/1 -> MATLAB Function/1
  MATLAB Function/1 -> Add1/1

== system vdynblksskidpad_final/Formula Student Vehicle/Simulink Physics - 7DOF/Powertrain & Driveline/Brakes and Wheels/scale factors with friction ==
  lamda_mu_x : Inport
  lamda_mu_y : Inport  Port=2
  0 : Constant  Value=[zeros(1,numWheels)]  VectorParams1D=off
  Reshape : Reshape  OutputDimensionality=Row vector (2-D)  OutputDimensions=[1,numWheels]
  Reshape1 : Reshape  OutputDimensionality=Row vector (2-D)  OutputDimensions=[1,numWheels]
  Signal Specification3 : SignalSpecification  Unit=1
  Vector Concatenate : Concatenate  NumInputs=5  Mode=Multidimensional array
  ones : Constant  Value=[ones(23,numWheels)]  VectorParams1D=off
  ones2 : Constant  Value=ones(1,numWheels)  VectorParams1D=off
  lambdas : Outport  Unit=1  VectorParamsAs1DForOutWhenUnconnected=off
  wires:
  lamda_mu_y/1 -> Reshape1/1
  lamda_mu_x/1 -> Reshape/1
  ones2/1 -> Vector Concatenate/1  "lambda_Fz0"
  Vector Concatenate/1 -> Signal Specification3/1
  ones/1 -> Vector Concatenate/5
  0/1 -> Vector Concatenate/4  "lamda_mu_V"
  Reshape1/1 -> Vector Concatenate/3
  Reshape/1 -> Vector Concatenate/2
  Signal Specification3/1 -> lambdas/1

== system vdynblksskidpad_final/Formula Student Vehicle/Simulink Physics - 7DOF/Powertrain & Driveline/Dual/Dual Fz ==
  In1 : Inport
  Bus Selector6 : BusSelector  OutputSignals=SuspWhlF
  Suspension_Vertical_Load : Gain  Gain=[0 0 1]  Multiplication=Matrix(K*u)
  Out1 : Outport  VectorParamsAs1DForOutWhenUnconnected=off
  wires:
  Suspension_Vertical_Load/1 -> Out1/1
  Bus Selector6/1 -> Suspension_Vertical_Load/1  "<SuspWhlF>"
  In1/1 -> Bus Selector6/1

== system vdynblksskidpad_final/Formula Student Vehicle/Simulink Physics - 7DOF/Powertrain & Driveline/Dual/Dual V ==
  In1 : Inport
  Bus Selector1 : BusSelector  OutputSignals=signal1.VehFdbk.BdyFrm.FrntAxl.Lft.Vel.xdot,signal1.VehFdbk.BdyFrm.FrntAxl.Lft.Vel.ydot,signal1.VehFdbk.BdyFrm.FrntAxl.Lft.Vel.zdot  OutputAsBus=on
  Bus Selector2 : BusSelector  OutputSignals=signal1.VehFdbk.BdyFrm.FrntAxl.Rght.Vel.xdot,signal1.VehFdbk.BdyFrm.FrntAxl.Rght.Vel.ydot,signal1.VehFdbk.BdyFrm.FrntAxl.Rght.Vel.zdot  OutputAsBus=on
  Bus Selector4 : BusSelector  OutputSignals=signal1.VehFdbk.BdyFrm.RearAxl.Lft.Vel.xdot,signal1.VehFdbk.BdyFrm.RearAxl.Lft.Vel.ydot,signal1.VehFdbk.BdyFrm.RearAxl.Lft.Vel.zdot  OutputAsBus=on
  Bus Selector5 : BusSelector  OutputSignals=signal1.VehFdbk.BdyFrm.RearAxl.Rght.Vel.xdot,signal1.VehFdbk.BdyFrm.RearAxl.Rght.Vel.ydot,signal1.VehFdbk.BdyFrm.RearAxl.Rght.Vel.zdot  OutputAsBus=on
  Bus to Vector{5..8} (4 alike) : BusToVector
  Vector Concatenate2 : Concatenate  NumInputs=4  Mode=Multidimensional array  ConcatenateDimension=2
  Out1 : Outport  VectorParamsAs1DForOutWhenUnconnected=off
  wires:
  Bus to Vector6/1 -> Vector Concatenate2/2
  Bus Selector2/1 -> Bus to Vector6/1
  Bus to Vector8/1 -> Vector Concatenate2/4
  Bus Selector4/1 -> Bus to Vector7/1
  Bus to Vector5/1 -> Vector Concatenate2/1
  Bus Selector1/1 -> Bus to Vector5/1
  Bus Selector5/1 -> Bus to Vector8/1
  Bus to Vector7/1 -> Vector Concatenate2/3
  Vector Concatenate2/1 -> Out1/1
  In1/1 -> Bus Selector1/1, Bus Selector2/1, Bus Selector4/1, Bus Selector5/1
